simulink model "CLVF"  (R2020a)
settings: Solver=FixedStepAuto  StartTime=0.0  StopTime=tsim  FixedStep=baseRate  RelTol=1e-3  EnableMultiTasking=on
values from neighbouring files (symbols this model uses):
  a = sqrt(sum(aTimesOVec.^2))    [Run_Initializer.m]    (also in a_max_CLVF2D.m = params(4))
  a_max = 0.4/BLACKMass    [Run_Initializer.m]
  a_prime = newParams(2)    [Run_Initializer.m]    (also in a_max_LVF.m = params(2))
  acceptableRadius = 0.05    [Run_Initializer.m]
  b = newParams(3)    [Run_Initializer.m]    (also in a_max_CLVF2D.m = params(3))
  baseRate = 0.05    [Run_Initializer.m]
  BLACKMass = model_param(3)    [Run_Initializer.m]
  d = [0.16;0.542;0]    [Run_Initializer.m]    (also in a_max_LVF.m = [rotStuff(3);rotStuff(4);rotStuff(5)])
  drop_states_BLACK = rC_I0    [Run_Initializer.m]
  drop_states_BLUE = [ xLength/2+0.9; yLength/2+0.5; 0]    [Run_Initializer.m]
  drop_states_RED = rT_I0    [Run_Initializer.m]
  F_thrusters_BLACK = 0.25.*ones(8,1)    [Run_Initializer.m]
  F_thrusters_BLUE = 0.25.*ones(8,1)    [Run_Initializer.m]
  F_thrusters_RED = 0.25.*ones(8,1)    [Run_Initializer.m]
  home_states_BLACK = [ xLength/2+0.4; yLength/2; 0]    [Run_Initializer.m]
  home_states_BLUE = [ xLength/2-0.9; yLength/2+0.5; 0]    [Run_Initializer.m]
  home_states_RED = [ xLength/2-0.4; yLength/2; 0]    [Run_Initializer.m]
  init_states_BLACK = rC_I0    [Run_Initializer.m]
  init_states_BLUE = [ xLength/2+0.9; yLength/2+0.5; 0]    [Run_Initializer.m]
  init_states_RED = rT_I0    [Run_Initializer.m]
  k_v_rel = 2*v_max/a_prime    (= 1)    [Run_Initializer.m]
  ka = newParams(2)    [Run_Initializer.m]    (also in a_max_CLVF2D.m = params(2))
  kc = newParams(1)    [Run_Initializer.m]    (also in a_max_CLVF2D.m = params(1))
  kd = 5.0    (= 5)    [Run_Initializer.m]
  Kd_tb = 0.4    [Run_Initializer.m]
  Kd_tblue = 0.4    [Run_Initializer.m]
  Kd_tr = 0.4    [Run_Initializer.m]
  Kd_xb = 5    [Run_Initializer.m]
  Kd_xblue = 5    [Run_Initializer.m]
  Kd_xr = 5    [Run_Initializer.m]
  Kd_yb = 5    [Run_Initializer.m]
  Kd_yblue = 5    [Run_Initializer.m]
  Kd_yr = 5    [Run_Initializer.m]
  Kp_tb = 0.1    [Run_Initializer.m]
  Kp_tblue = 0.1    [Run_Initializer.m]
  Kp_tr = 0.1    [Run_Initializer.m]
  Kp_xb = 2    [Run_Initializer.m]
  Kp_xblue = 2    [Run_Initializer.m]
  Kp_xr = 2    [Run_Initializer.m]
  Kp_yb = 2    [Run_Initializer.m]
  Kp_yblue = 2    [Run_Initializer.m]
  Kp_yr = 2    [Run_Initializer.m]
  noise_variance_BLACK = 0    [Run_Initializer.m]
  noise_variance_BLUE = 0    [Run_Initializer.m]
  noise_variance_RED = 0    [Run_Initializer.m]
  o_hat_B = aTimesOVec./a    [Run_Initializer.m]
  o_hat_prime = o_prime/sqrt(sum(o_prime.^2))    [Run_Initializer.m]
  Phase0_End = Phase0_Duration    (= 10)    [Run_Initializer.m]
  Phase1_End = Phase0_Duration + Phase1_Duration    (= 15)    [Run_Initializer.m]
  Phase2_End = Phase0_Duration + Phase1_Duration +                                   Phase2_Duration    (= 35)    [Run_Initializer.m]
  Phase3_End = Phase0_Duration + Phase1_Duration +                                   Phase2_Duration + Phase3_Duration    [Run_Initializer.m]
  Phase3_SubPhase1_End = Phase2_End + Phase3_SubPhase1_Duration    (= 40)    [Run_Initializer.m]
  Phase3_SubPhase2_End = Phase2_End + Phase3_SubPhase1_Duration +                                   Phase3_SubPhase2_Duration    (= 45)    [Run_Initializer.m]
  Phase3_SubPhase3_End_BLACK = Phase2_End + Phase3_SubPhase1_Duration +                                   Phase3_SubPhase2_Duration +                                  Phase3_SubPhase3_Duration + Phase3_SubPhase3_and_a_half    (= 51)    [Run_Initializer.m]
  Phase3_SubPhase3_End_RED = Phase2_End + Phase3_SubPhase1_Duration +                                   Phase3_SubPhase2_Duration +                                  Phase3_SubPhase3_Duration    (= 46)    [Run_Initializer.m]
  Phase3_SubPhase4_End = Phase2_End + Phase3_SubPhase1_Duration +                                   Phase3_SubPhase2_Duration +                                  Phase3_SubPhase3_Duration +                                  Phase3_SubPhase4_Duration + Phase3_SubPhase3_and_a_half    [Run_Initializer.m]
  Phase4_End = Phase0_Duration + Phase1_Duration +                                   Phase2_Duration + Phase3_Duration +                                   Phase4_Duration    [Run_Initializer.m]
  Phase5_End = Phase0_Duration + Phase1_Duration +                                   Phase2_Duration + Phase3_Duration +                                   Phase4_Duration + Phase5_Duration    [Run_Initializer.m]
  r_co = r_co_over_a_prime*a_prime    (= 0.16)    [Run_Initializer.m]
  rC_I0 = [0.9*xLength;yLength/2-0.5;pi/2]    [Run_Initializer.m]
  rT_I0 = [yLength/2;yLength/2;possibleStarts(startingRotation)]    [Run_Initializer.m]
  serverRate = 0.1    [Run_Initializer.m]
  sys_BLACK = c2d(sys_BLACK_CONT, baseRate)    [Run_Initializer.m]
  sys_BLACK_ROT = c2d(sys_BLACK_rot_CONT, baseRate)    [Run_Initializer.m]
  sys_RED = c2d(sys_RED_CONT, baseRate)    [Run_Initializer.m]
  sys_RED_ROT = c2d(sys_RED_rot_CONT, baseRate)    [Run_Initializer.m]
  theta_d = 30*d2r    (= 0.523598775598)    [Run_Initializer.m]    (also in a_max_LVF.m = rotStuff(2))
  thruster_dist2CG_BLACK = [83.42;-52.58;55.94;-60.05;54.08;-53.92;77.06;-55.94]    [Run_Initializer.m]
  thruster_dist2CG_BLUE = [83.42;-52.58;55.94;-60.05;54.08;-53.92;77.06;-55.94]    [Run_Initializer.m]
  thruster_dist2CG_RED = [49.92;-78.08;70.46;-63.54;81.08;-50.42;57.44;-75.96]    [Run_Initializer.m]
  w_body = 6.0 * d2r    (= 0.10471975512)    [Run_Initializer.m]
undefined symbols (not defined in the file or in its folder): DiscIntNeverNeededParam, Discrete, Phase3_SubPhase3_End, platformSelection, simMode, Time, WhoAmI
libraries: dspstat3 x18, dspsigops x14, raspberrypiBasiclib x10, embdlinuxlib x8, simulink x8, ctrlSharedLib x4, mspfiltlib x3, dsparch4 x3, dspswit3 x2, MainLibrary x2, sensehatlib x1
(part 10 of 10)

== matlab function CLVF/Phase #2: Move to Initial Position/Change BLUE Behavior/Hough Control/MATLAB Function4 ==
  data: Oy input; e_out output; e_in input
function e_out = fcn(Oy, e_in)

a = sign(Oy'*e_in);
e_out = -a*norm(e_in);

== matlab function CLVF/Phase #3: Experiment/Change BLACK Behavior/Sub-Phase #4/Lyapunov GNC/Navigation/tau_km1_RED/MATLAB Function ==
  data: TIME input; y output; SERVER input
function y = fcn(TIME, SERVER)

if mod(TIME,SERVER) == 0
    y = 1;
else
    y = 0;
end

== matlab function CLVF/Phase #3: Experiment/Change BLACK Behavior/Sub-Phase #4/Lyapunov GNC/Navigation/u_km1_BLACK/MATLAB Function ==
  data: TIME input; y output; SERVER input
function y = fcn(TIME, SERVER)

if mod(TIME,SERVER) == 0
    y = 1;
else
    y = 0;
end

== matlab function CLVF/Phase #3: Experiment/Change BLACK Behavior/Sub-Phase #4/Lyapunov GNC/Navigation/u_km1_RED/MATLAB Function ==
  data: TIME input; y output; SERVER input
function y = fcn(TIME, SERVER)

if mod(TIME,SERVER) == 0
    y = 1;
else
    y = 0;
end

== matlab function CLVF/Phase #3: Experiment/Change BLACK Behavior/Sub-Phase #4/Lyapunov GNC/P + FF Controller ==
  data: h input; f output; vC_I input; a_ff input; BLACKMass parameter; kd parameter
function f = fcn(h, vC_I, a_ff, BLACKMass, kd)

f = kd*(h - vC_I) + BLACKMass*a_ff;
end

== matlab function CLVF/Phase #3: Experiment/Change BLUE Behavior/Sub-Phase #1/Hough Control/MATLAB Function2 ==
  data: Oy output; z input; Ox output
function [Oy, Ox]   = C3( z )
%C3 gives the rotation matrix about the z-axis for an angle 'z'
%   z - the angle about the z-axis which you rotate
%   A - the rotation matrix

Ox = [cos(z) sin(z); -sin(z) cos(z)]*[1;0];
Oy = [cos(z) sin(z); -sin(z) cos(z)]*[0;1];
end

== matlab function CLVF/Simulate Plant Dynamics/BLUE  Dynamics Model/MATLAB Function ==
  data: control_inputs input; x_ddot output; model_param parameter
function x_ddot = BLUE_dynamics(control_inputs, model_param)

%#codegen
% Fully define the size of x_ddot() for code generation:
x_ddot     = zeros(3,1);

% Extract the servicer model parameters from the model_param vector defined
% in initialize.m:
m_BLUE    = model_param(5);
I_BLUE    = model_param(6);

% Extract the control inputs from the control_input vector:
Fx        = control_inputs(1);              % [N]
Fy        = control_inputs(2);              % [N]
Tz        = control_inputs(3);              % [N.m]

% Calculate the state acceleration vector:
x_ddot(1) = Fx/m_BLUE;                      % [m/s^2]
x_ddot(2) = Fy/m_BLUE;                      % [m/s^2]
x_ddot(3) = Tz/I_BLUE;                      % [rad/s^2]

end

== matlab function CLVF/Phase #3: Experiment/Change BLUE Behavior/Sub-Phase #1/Hough Control/MATLAB Function3 ==
  data: z input; Ox output
function Ox    = C3( z )
%C3 gives the rotation matrix about the z-axis for an angle 'z'
%   z - the angle about the z-axis which you rotate
%   A - the rotation matrix

Ox = [cos(z) sin(z); -sin(z) cos(z)]*[1;0];
end

== matlab function CLVF/Phase #3: Experiment/Change BLUE Behavior/Sub-Phase #1/Hough Control/MATLAB Function4 ==
  data: Oy input; e_out output; e_in input
function e_out = fcn(Oy, e_in)

a = sign(Oy'*e_in);
e_out = -a*norm(e_in);

== matlab function CLVF/Phase #3: Experiment/Change BLUE Behavior/Sub-Phase #4/Hough Control/MATLAB Function2 ==
  data: Oy output; z input; Ox output
function [Oy, Ox]   = C3( z )
%C3 gives the rotation matrix about the z-axis for an angle 'z'
%   z - the angle about the z-axis which you rotate
%   A - the rotation matrix

Ox = [cos(z) sin(z); -sin(z) cos(z)]*[1;0];
Oy = [cos(z) sin(z); -sin(z) cos(z)]*[0;1];
end

== matlab function CLVF/Phase #3: Experiment/Change RED Behavior/Sub-Phase #1/Hough Control/MATLAB Function2 ==
  data: Oy output; z input; Ox output
function [Oy, Ox]   = C3( z )
%C3 gives the rotation matrix about the z-axis for an angle 'z'
%   z - the angle about the z-axis which you rotate
%   A - the rotation matrix

Ox = [cos(z) sin(z); -sin(z) cos(z)]*[1;0];
Oy = [cos(z) sin(z); -sin(z) cos(z)]*[0;1];
end

== matlab function CLVF/Phase #3: Experiment/Change RED Behavior/Sub-Phase #1/Hough Control/MATLAB Function3 ==
  data: z input; Ox output
function Ox    = C3( z )
%C3 gives the rotation matrix about the z-axis for an angle 'z'
%   z - the angle about the z-axis which you rotate
%   A - the rotation matrix

Ox = [cos(z) sin(z); -sin(z) cos(z)]*[1;0];
end

== matlab function CLVF/Phase #3: Experiment/Change BLACK Behavior/Sub-Phase #4/Hough Control/MATLAB Function4 ==
  data: Oy input; e_out output; e_in input
function e_out = fcn(Oy, e_in)

a = sign(Oy'*e_in);
e_out = -a*norm(e_in);

== matlab function CLVF/Phase #3: Experiment/Change BLACK Behavior/Sub-Phase #1/Hough Control/MATLAB Function2 ==
  data: Oy output; z input; Ox output
function [Oy, Ox]   = C3( z )
%C3 gives the rotation matrix about the z-axis for an angle 'z'
%   z - the angle about the z-axis which you rotate
%   A - the rotation matrix

Ox = [cos(z) sin(z); -sin(z) cos(z)]*[1;0];
Oy = [cos(z) sin(z); -sin(z) cos(z)]*[0;1];
end

== matlab function CLVF/Phase #3: Experiment/Change BLACK Behavior/Sub-Phase #1/Hough Control/MATLAB Function3 ==
  data: z input; Ox output
function Ox    = C3( z )
%C3 gives the rotation matrix about the z-axis for an angle 'z'
%   z - the angle about the z-axis which you rotate
%   A - the rotation matrix

Ox = [cos(z) sin(z); -sin(z) cos(z)]*[1;0];
end

== matlab function CLVF/Phase #3: Experiment/Change BLACK Behavior/Sub-Phase #1/Hough Control/MATLAB Function4 ==
  data: Oy input; e_out output; e_in input
function e_out = fcn(Oy, e_in)

a = sign(Oy'*e_in);
e_out = -a*norm(e_in);

== matlab function CLVF/Phase #3: Experiment/Change BLUE Behavior/Sub-Phase #4/Hough Control/MATLAB Function3 ==
  data: z input; Ox output
function Ox    = C3( z )
%C3 gives the rotation matrix about the z-axis for an angle 'z'
%   z - the angle about the z-axis which you rotate
%   A - the rotation matrix

Ox = [cos(z) sin(z); -sin(z) cos(z)]*[1;0];
end

== matlab function CLVF/Simulate Plant Dynamics/RED Dynamics Model/MATLAB Function ==
  data: control_inputs input; x_ddot output; model_param parameter
function x_ddot = RED_dynamics(control_inputs, model_param)

%#codegen
% Fully define the size of x_ddot() for code generation:
x_ddot     = zeros(3,1);

% Extract the servicer model parameters from the model_param vector defined
% in initialize.m:
m_RED    = model_param(1);
I_RED    = model_param(2);

% Extract the control inputs from the control_input vector:
Fx        = control_inputs(1);              % [N]
Fy        = control_inputs(2);              % [N]
Tz        = control_inputs(3);              % [N.m]

% Calculate the state acceleration vector:
x_ddot(1) = Fx/m_RED;                      % [m/s^2]
x_ddot(2) = Fy/m_RED;                      % [m/s^2]
x_ddot(3) = Tz/I_RED;                      % [rad/s^2]

end

== matlab function CLVF/Phase #3: Experiment/Change BLUE Behavior/Sub-Phase #4/Hough Control/MATLAB Function4 ==
  data: Oy input; e_out output; e_in input
function e_out = fcn(Oy, e_in)

a = sign(Oy'*e_in);
e_out = -a*norm(e_in);

== matlab function CLVF/Phase #5: Hold Home/Change BLACK Behavior/Hough Control/MATLAB Function2 ==
  data: Oy output; z input; Ox output
function [Oy, Ox]   = C3( z )
%C3 gives the rotation matrix about the z-axis for an angle 'z'
%   z - the angle about the z-axis which you rotate
%   A - the rotation matrix

Ox = [cos(z) sin(z); -sin(z) cos(z)]*[1;0];
Oy = [cos(z) sin(z); -sin(z) cos(z)]*[0;1];
end

== matlab function CLVF/Phase #5: Hold Home/Change BLACK Behavior/Hough Control/MATLAB Function3 ==
  data: z input; Ox output
function Ox    = C3( z )
%C3 gives the rotation matrix about the z-axis for an angle 'z'
%   z - the angle about the z-axis which you rotate
%   A - the rotation matrix

Ox = [cos(z) sin(z); -sin(z) cos(z)]*[1;0];
end

== matlab function CLVF/Phase #5: Hold Home/Change BLACK Behavior/Hough Control/MATLAB Function4 ==
  data: Oy input; e_out output; e_in input
function e_out = fcn(Oy, e_in)

a = sign(Oy'*e_in);
e_out = -a*norm(e_in);

== matlab function CLVF/Phase #4: Return Home/Change BLUE Behavior/Hough Control/MATLAB Function2 ==
  data: Oy output; z input; Ox output
function [Oy, Ox]   = C3( z )
%C3 gives the rotation matrix about the z-axis for an angle 'z'
%   z - the angle about the z-axis which you rotate
%   A - the rotation matrix

Ox = [cos(z) sin(z); -sin(z) cos(z)]*[1;0];
Oy = [cos(z) sin(z); -sin(z) cos(z)]*[0;1];
end

== matlab function CLVF/Phase #4: Return Home/Change BLUE Behavior/Hough Control/MATLAB Function3 ==
  data: z input; Ox output
function Ox    = C3( z )
%C3 gives the rotation matrix about the z-axis for an angle 'z'
%   z - the angle about the z-axis which you rotate
%   A - the rotation matrix

Ox = [cos(z) sin(z); -sin(z) cos(z)]*[1;0];
end

== matlab function CLVF/Phase #4: Return Home/Change BLUE Behavior/Hough Control/MATLAB Function4 ==
  data: Oy input; e_out output; e_in input
function e_out = fcn(Oy, e_in)

a = sign(Oy'*e_in);
e_out = -a*norm(e_in);

== matlab function CLVF/Phase #5: Hold Home/Change RED Behavior/Hough Control/MATLAB Function2 ==
  data: Oy output; z input; Ox output
function [Oy, Ox]   = C3( z )
%C3 gives the rotation matrix about the z-axis for an angle 'z'
%   z - the angle about the z-axis which you rotate
%   A - the rotation matrix

Ox = [cos(z) sin(z); -sin(z) cos(z)]*[1;0];
Oy = [cos(z) sin(z); -sin(z) cos(z)]*[0;1];
end

== matlab function CLVF/Phase #5: Hold Home/Change RED Behavior/Hough Control/MATLAB Function3 ==
  data: z input; Ox output
function Ox    = C3( z )
%C3 gives the rotation matrix about the z-axis for an angle 'z'
%   z - the angle about the z-axis which you rotate
%   A - the rotation matrix

Ox = [cos(z) sin(z); -sin(z) cos(z)]*[1;0];
end

== matlab function CLVF/Phase #5: Hold Home/Change RED Behavior/Hough Control/MATLAB Function4 ==
  data: Oy input; e_out output; e_in input
function e_out = fcn(Oy, e_in)

a = sign(Oy'*e_in);
e_out = -a*norm(e_in);

== matlab function CLVF/Phase #5: Hold Home/Change BLUE Behavior/Hough Control/MATLAB Function2 ==
  data: Oy output; z input; Ox output
function [Oy, Ox]   = C3( z )
%C3 gives the rotation matrix about the z-axis for an angle 'z'
%   z - the angle about the z-axis which you rotate
%   A - the rotation matrix

Ox = [cos(z) sin(z); -sin(z) cos(z)]*[1;0];
Oy = [cos(z) sin(z); -sin(z) cos(z)]*[0;1];
end

== matlab function CLVF/Simulate Plant Dynamics/BLACK Dynamics Model/MATLAB Function ==
  data: control_inputs input; x_ddot output; model_param parameter
function x_ddot = BLACK_dynamics(control_inputs, model_param)

%#codegen
% Fully define the size of x_ddot() for code generation:
x_ddot     = zeros(3,1);

% Extract the servicer model parameters from the model_param vector defined
% in initialize.m:
m_BLACK    = model_param(3);
I_BLACK    = model_param(4);

% Extract the control inputs from the control_input vector:
Fx        = control_inputs(1);              % [N]
Fy        = control_inputs(2);              % [N]
Tz        = control_inputs(3);              % [N.m]

% Calculate the state acceleration vector:
x_ddot(1) = Fx/m_BLACK;                      % [m/s^2]
x_ddot(2) = Fy/m_BLACK;                      % [m/s^2]
x_ddot(3) = Tz/I_BLACK;                      % [rad/s^2]

end

== matlab function CLVF/Phase #5: Hold Home/Change BLUE Behavior/Hough Control/MATLAB Function3 ==
  data: z input; Ox output
function Ox    = C3( z )
%C3 gives the rotation matrix about the z-axis for an angle 'z'
%   z - the angle about the z-axis which you rotate
%   A - the rotation matrix

Ox = [cos(z) sin(z); -sin(z) cos(z)]*[1;0];
end

== matlab function CLVF/Phase #5: Hold Home/Change BLUE Behavior/Hough Control/MATLAB Function4 ==
  data: Oy input; e_out output; e_in input
function e_out = fcn(Oy, e_in)

a = sign(Oy'*e_in);
e_out = -a*norm(e_in);

== matlab function CLVF/From Torque, Command RW/Change RED Behavior/Calculate Saturated RPM Signal/Calculate RW RPM Increment ==
  data: Tz_Sat input; dRPM_RW output
function dRPM_RW = Calc_RW_RPM(Tz_Sat)

dRPM_RW =  (Tz_Sat/0.007244720)*(60/2/pi)*0.1;

end

== matlab function CLVF/From Torque, Command RW/Change RED Behavior/Wheel RPM to PWM/Check if RW is Ready ==
  data: Status input; EnableSig output; WheelRPM_In input; WheelRPM_Out output
function [EnableSig, WheelRPM_Out] = Check_Wheel_Status(Status, WheelRPM_In)

if Status == 0
    EnableSig    = 1;
    WheelRPM_Out = WheelRPM_In;
else
    EnableSig    = 0;
    WheelRPM_Out = 0;
end

end

== matlab function CLVF/From Torque, Command RW/Change RED Behavior/Wheel RPM to PWM/Get RW Direction ==
  data: MotorRPM_Sat input; WheelDirection output
function WheelDirection = GetDirection(MotorRPM_Sat)

if MotorRPM_Sat > 0
    WheelDirection = 0;
else
    WheelDirection = 1;
end
        
end

== matlab function CLVF/From Torque, Command RW/Change RED Behavior/Wheel RPM to PWM/RPM to PWM Value ==
  data: MotorRPM_Sat input; MotorPWM output
function MotorPWM = RPM2PWM(MotorRPM_Sat)

PWMRange = 0.9-0.1;

MotorPWM = ((MotorRPM_Sat*PWMRange)/7000) + 0.1;

end

== matlab function CLVF/Phase #3: Experiment/Change BLACK Behavior/Sub-Phase #4/Lyapunov GNC/CLVF Approach/CLVF Guidance ==
  data: rC_T input; h output; vC_T input; vT_I input; aT_I input; theta input; theta_dot input; theta_ddot input; a_ff output; r output; alignmentAngle output; o_hat_B parameter; a parameter; b parameter; ka parameter; kc parameter; o_hat output
function [h, a_ff, r, alignmentAngle, o_hat] = fcn(rC_T, vC_T, vT_I, aT_I, theta, theta_dot, theta_ddot, o_hat_B, a, b, ka, kc)
    
    % Prep some of the variables for inclusion into the CLVF function:
        
        o_hat = C3(theta)'*o_hat_B;
        
        w_OI = [0;0;theta_dot];
        w_dot_OI = [0;0;theta_ddot];
        
        q = 0.0000001; % Small number!

                
        
[h, a_ff, r, alignmentAngle] = CLVF2(rC_T, w_OI, w_dot_OI, o_hat, vT_I, aT_I, a, b, ka, kc, vC_T,q);

== matlab function CLVF/Phase #3: Experiment/Change BLACK Behavior/Sub-Phase #4/Lyapunov GNC/Lyapunov/Body-Fixed Guidance ==
  data: rC_T input; hC_T output; theta input; theta_dot input; k_v_rel parameter; d parameter; o_hat_prime parameter; theta_d parameter; a_prime parameter; acc_ff output; theta_ddot input; r output; newTheta output; vT_I input; o_hat output; r_co parameter; vC_T input
function [hC_T, acc_ff, r, newTheta, o_hat] = lyapVecField(rC_T, theta, theta_dot, k_v_rel, d, o_hat_prime, theta_d, a_prime, theta_ddot, vT_I, r_co, vC_T)

    C_BIt = C3(theta);
    C_IB = C_BIt';
    
    w_OI = [0;0;theta_dot];
    w_dot_OI = [0;0;theta_ddot];
    
    o_hat = C_IB * o_hat_prime;
    
    % The velocity of the "target" is actually the velocity of the docking
    % port!
        vD_I = vT_I + skew(w_OI)*(C_IB * d);
        vC_D = vC_T - skew(w_OI)*(C_IB * d);
        
    % The position relative to the target is actaully the position relative
    % to the docking port:
        rD_T = C_IB*d;
        rC_D = rC_T - rD_T;
        
    % The acceleration of the target is just the acceleration of the
    % docking port:
        aD_I = -theta_dot^2*C_IB * d; % Assuming that omega_dot == 0.
    
    % w_dot = [0;0;theta_ddot]; Will be needed for the acc_ff
    
        q = 0.0001; % Small number!

    [hC_T, acc_ff, r, newTheta] = LVF(rC_D, o_hat, q, k_v_rel, theta_d, w_OI, vD_I, a_prime, r_co, vC_D, aD_I, w_dot_OI);
    
end

== matlab function CLVF/Simulate Plant Dynamics/Sample and Hold Data to Match PhaseSpace (BLUE)/MATLAB Function ==
  data: TIME input; y output; SERVER input
function y = fcn(TIME, SERVER)

if mod(TIME,SERVER) == 0
    y = 1;
else
    y = 0;
end

== matlab function CLVF/Phase #3: Experiment/Change BLACK Behavior/Sub-Phase #4/Lyapunov GNC/Navigation/tau_km1_BLACK/MATLAB Function ==
  data: TIME input; y output; SERVER input
function y = fcn(TIME, SERVER)

if mod(TIME,SERVER) == 0
    y = 1;
else
    y = 0;
end

== matlab function CLVF/Gyroscope & Acceleration Algorithms/Change RED Behavior/Create Rotation Matrix ==
  data: Rz input; C_Ib output
function C_Ib = RotateFrame(Rz)

C_bI = [  cos(Rz) sin(Rz)
         -sin(Rz) cos(Rz) ];

C_Ib = inv(C_bI);

end

== matlab function CLVF/Gyroscope & Acceleration Algorithms/Change BLACK Behavior/Create Rotation Matrix ==
  data: Rz input; C_Ib output
function C_Ib = RotateFrame(Rz)

C_bI = [  cos(Rz) sin(Rz)
         -sin(Rz) cos(Rz) ];

C_Ib = inv(C_bI);

end

== matlab function CLVF/Gyroscope & Acceleration Algorithms/Change RED Behavior/ChangeOrientation ==
  data: u input; y output
function y = ChangeOrientation(u)

y = rotz(-90)*u';

== matlab function CLVF/Gyroscope & Acceleration Algorithms/Change BLACK Behavior/ChangeOrientation ==
  data: u input; y output
function y = ChangeOrientation(u)

y = rotz(-90)*u';

== matlab function CLVF/Gyroscope & Acceleration Algorithms/Change BLUE Behavior/ChangeOrientation ==
  data: u input; y output
function y = ChangeOrientation(u)

y = rotz(-90)*u';

== matlab function CLVF/Gyroscope & Acceleration Algorithms/Change BLUE Behavior/Create Rotation Matrix ==
  data: Rz input; C_Ib output
function C_Ib = RotateFrame(Rz)

C_bI = [  cos(Rz) sin(Rz)
         -sin(Rz) cos(Rz) ];

C_Ib = inv(C_bI);

end

== matlab function CLVF/Phase #3: Experiment/Change BLACK Behavior/Sub-Phase #4/Lyapunov GNC/SWITCH/inDesiredRadius ==
  data: rC_T input; newCnt output; theta input; currentCnt input; o_hat_B parameter; a parameter; acceptableRadius parameter
function newCnt = accumulateTimeInRadius(rC_T, theta, currentCnt, o_hat_B, a, acceptableRadius)

% Check whether we are in the acceptable radius
        desiredPosition = C3(theta)' * o_hat_B * a;
        positionError = sqrt((desiredPosition - rC_T)'*(desiredPosition - rC_T));
        
        if positionError <= acceptableRadius
            newCnt = currentCnt+1;
        else
            newCnt = 0; % Reset
        end

end

== matlab function CLVF/Phase #3: Experiment/Change BLACK Behavior/Sub-Phase #4/Lyapunov GNC/SWITCH/sufficientTime ==
  data: oneOrZero output; cnt input; cntThreshold parameter
function oneOrZero = fcn(cnt, cntThreshold)

    if cnt < cntThreshold
        oneOrZero = 0; % Not enough.
    else
        oneOrZero = 1;
    end
end

== matlab function CLVF/From Force//Torque to PWM Signal/Change BLUE Behavior/Calculate Thruster ON//OFF/MATLAB Function ==
  data: H output; thruster_dist2CG_BLUE parameter; F_thrusters_BLUE parameter
function H = MakeH(thruster_dist2CG_BLUE,F_thrusters_BLUE)

Vec1 = [ -1
         -1
          0 
          0
          1
          1
          0
          0 ];
      
Vec2 = [  0
          0
          1
          1
          0
          0
         -1
         -1 ];
     
Vec3 = thruster_dist2CG_BLUE./1000;

Mat1 = [Vec1, Vec2, Vec3]';

Mat2 = diag((F_thrusters_BLUE./2));

H    = Mat1*Mat2;

end

== matlab function CLVF/Phase #3: Experiment/Change BLACK Behavior/Sub-Phase #4/Lyapunov GNC/getMag ==
  data: u input; y output
function y = fcn(u)

y = sqrt(sum(u.^2));

== matlab function CLVF/Phase #3: Experiment/Change BLACK Behavior/Sub-Phase #4/Lyapunov GNC/getNorm ==
  data: u input; y output
function y = fcn(u)

y = sqrt(sum(u.^2));

== matlab function CLVF/Phase #3: Experiment/Change BLACK Behavior/Sub-Phase #4/States in Target-Fixed Frame/MATLAB Function ==
  data: d_T output; theta_T input; d parameter
function d_T = fcn(theta_T, d)

    d_T = C3(theta_T)'*d;
    
end

== matlab function CLVF/Phase #3: Experiment/Change BLACK Behavior/Sub-Phase #4/getDesiredRotation ==
  data: rC_D input; thetaC output; o_hat_dock input; whichField input
function thetaC = fcn(rC_D, o_hat_dock, whichField)

    rD_C = -rC_D;

    if whichField == 0 % The CLVF:
        thetaC = atan2(rD_C(2),rD_C(1)) - pi/2;
    else
        o_hat_opposite = -o_hat_dock;
        thetaC = atan2(o_hat_opposite(2), o_hat_opposite(1)) - pi/2;
    end

end

== matlab function CLVF/Phase #3: Experiment/Change RED Behavior/Sub-Phase #1/Hough Control/MATLAB Function4 ==
  data: Oy input; e_out output; e_in input
function e_out = fcn(Oy, e_in)

a = sign(Oy'*e_in);
e_out = -a*norm(e_in);

== matlab function CLVF/Phase #3: Experiment/Change RED Behavior/Sub-Phase #4/Hough Control/MATLAB Function2 ==
  data: Oy output; z input; Ox output
function [Oy, Ox]   = C3( z )
%C3 gives the rotation matrix about the z-axis for an angle 'z'
%   z - the angle about the z-axis which you rotate
%   A - the rotation matrix

Ox = [cos(z) sin(z); -sin(z) cos(z)]*[1;0];
Oy = [cos(z) sin(z); -sin(z) cos(z)]*[0;1];
end

== matlab function CLVF/Phase #3: Experiment/Change RED Behavior/Sub-Phase #4/Hough Control/MATLAB Function3 ==
  data: z input; Ox output
function Ox    = C3( z )
%C3 gives the rotation matrix about the z-axis for an angle 'z'
%   z - the angle about the z-axis which you rotate
%   A - the rotation matrix

Ox = [cos(z) sin(z); -sin(z) cos(z)]*[1;0];
end

== matlab function CLVF/Phase #3: Experiment/Change RED Behavior/Sub-Phase #4/Hough Control/MATLAB Function4 ==
  data: Oy input; e_out output; e_in input
function e_out = fcn(Oy, e_in)

a = sign(Oy'*e_in);
e_out = -a*norm(e_in);

== matlab function CLVF/From Force//Torque to PWM Signal/Change BLUE Behavior/Calculate Thruster ON//OFF/MATLAB Function1 ==
  data: H output; thruster_dist2CG_BLUE parameter; F_thrusters_BLUE parameter
function H = MakeH(thruster_dist2CG_BLUE,F_thrusters_BLUE)

Vec1 = [ -1
         -1
          0 
          0
          1
          1
          0
          0 ];
      
Vec2 = [  0
          0
          1
          1
          0
          0
         -1
         -1 ];
     
Vec3 = thruster_dist2CG_BLUE./1000;

Mat1 = [Vec1, Vec2, Vec3]';

Mat2 = diag((F_thrusters_BLUE./2));

H    = Mat1*Mat2;

end

== matlab function CLVF/From Force//Torque to PWM Signal/Change BLUE Behavior/Calculate Thruster ON//OFF/MATLAB Function2 ==
  data: ThrustPer_Final output; ThrustPer input
function ThrustPer_Final  = ThrusterSat(ThrustPer)

ValveTime       = 0.007;
TControl        = 0.1;
ThrustPer_Final = zeros(8,1);

if max(ThrustPer) > 1
    ThrustPer_Sat = ThrustPer/max(ThrustPer);
else
    ThrustPer_Sat = ThrustPer;
end

for i = 1:8
    if ThrustPer_Sat(i) > ValveTime/TControl 
        ThrustPer_Final(i) = ThrustPer_Sat(i);
    else
        ThrustPer_Final(i) = 0;
    end
end
   

end

== matlab function CLVF/From Force//Torque to PWM Signal/Change BLUE Behavior/Calculate Thruster ON//OFF/Rotate Forces to Inertial/Create Rotation Matrix ==
  data: Rz input; C_Ib output
function C_Ib = RotateFrame(Rz)

C_bI = [  cos(Rz) sin(Rz)
         -sin(Rz) cos(Rz) ];

C_Ib = inv(C_bI);

end

== matlab function CLVF/From Force//Torque to PWM Signal/Change BLUE Behavior/Rotate Forces to Body/Create Rotation Matrix ==
  data: Rz input; C_bI output
function C_bI = RotateFrame(Rz)

C_bI = [  cos(Rz) sin(Rz)
         -sin(Rz) cos(Rz) ];

end
